simulink model "ASM_Traffic"  (R2026a)
settings: Solver=ode1  StartTime=SIM.tstart.v  StopTime=SIM.tend.v  FixedStep=SIM.StepSize.v
PostLoadFcn:
  | if any(exist('dsrtsu_mdlpostloadfcn', 'file') ~= 0), dsrtsu_mdlpostloadfcn('Execute', bdroot); end
  | try, asm_mdl_postloadfcn(bdroot, 'UpdateModel', 3600); catch, disp(lasterr); end,
InitFcn:
  | , if any(exist('rtifpga_mdlclblib', 'file') ~= 0), rtifpga_mdlclblib('Init', bdroot); end,
  | , if any(exist('dsmpb_private', 'file') ~= 0), dsmpb_private('dsmpb_mdlclblib', 'Init', bdroot); end,
model workspace (MAT data in the model file):
  asmReferencePath = [0 0.01 0.02 0.03 0.04 0.05 0.06 0.07 0.08 0.09 0.1 0.11 ... (350007 elements, 50001x7)]
  roadBounds : Simulink.Parameter (value not decoded)
  safetyAxes : Simulink.Parameter (value not decoded)
undefined symbols (not defined in the file): _to_, a0b2, ASM_BrakeHydraulics_DemoSystems, ASM_VehicleDynamics_DemoSystems, b98103fe8ad365046cd0, BrakeCircuit, controllerConfig, CPT, Crankshaft, DiscIntNeverNeededParam, dsmsi, FinalDriveAssembly, MDL, ModeSignals, mu, Pos_BrakePedal_Maneuver, rad, RefSignals, roadFamilyData, roadFamilyId, s_to_rpm, SIM, SoftECU, Suspension, Tire, Transmission
libraries: ASM_Traffic_lib x135, simulink x98, ASM_Utils_lib x77, ASM_VehicleDynamics_lib x70, ASM_Environment_lib x22, dsmpblib x20, dsmsilib x15, MDLD_Utils_lib x10, ASM_BrakeHydraulics_lib x3, sl_discontinuities x2
(part 41 of 65)

== system ASM_Traffic/Environment/Sensors/PlantModel/Object_Sensor_2D/SensorParameters ==
  2D_Sensors_Common_Signals : Subsystem
  Bus Creator : BusCreator  Inputs=8
  Demux{,1..6} (7 alike) : Demux  Outputs=3
  Mux{1..7} (7 alike) : Mux  Inputs=14
  OBJECT_SENSOR_2D_PARAMETERS_1 : ASM_Traffic_lib/Sensors/Object_Sensor_2D/OBJECT_SENSOR_2D_PARAMETERS  Tag=ASM_SUBCOMPONENT  Sw_Sensor_Enable=MDL.Traffic.Sensors.ObjectSensor2D_1.Sw_Sensor_Enable  Const_SensorIdx=MDL.Traffic.Sensors.ObjectSensor2D_1.Const_SensorIdx  Const_t_Offs_Sensor=MDL.Traffic.Sensors.ObjectSensor2D_1.Const_t_Offs_Sensor  Const_t_Cycle_Sensor=MDL.Traffic.Sensors.ObjectSensor2D_1.Const_t_Cycle_Sensor  Const_t_Delay_SensorOutput=MDL.Traffic.Sensors.ObjectSensor2D_1.Const_t_Delay_SensorOutput  Const_Pos_Sensor_Apex_CoorSys_V=MDL.Traffic.Sensors.ObjectSensor2D_1.Const_Pos_Sensor_Apex_CoorSys_V  Const_Angle_z_Orientation_Sensor_CoorSys_V=MDL.Traffic.Sensors.ObjectSensor2D_1.Const_Angle_z_Orientation_Sensor_CoorSys_V  Const_Angle_ScopeZone_Horizontal=MDL.Traffic.Sensors.ObjectSensor2D_1.Const_Angle_ScopeZone_Horizontal  Const_Length_ScopeZone=MDL.Traffic.Sensors.ObjectSensor2D_1.Const_Length_ScopeZone  Const_Num_SensorRays_Used=MDL.Traffic.Sensors.ObjectSensor2D_1.Const_Num_SensorRays_Used  Sw_Sensor_Detection_Mode=MDL.Traffic.Sensors.ObjectSensor2D_1.Sw_Sensor_Detection_Mode  Sw_Object_Detection_Mode=MDL.Traffic.Sensors.ObjectSensor2D_1.Sw_Object_Detection_Mode  ASMProperties=struct('Name','OBJECT_SENSOR_2D_PARAMETERS','Version','5.0','Library','ASM_Traffic_lib')  ASMInstanceName=object_sensor_2d_parameters  ASMInstanceID=1
  OBJECT_SENSOR_2D_PARAMETERS_2 : ASM_Traffic_lib/Sensors/Object_Sensor_2D/OBJECT_SENSOR_2D_PARAMETERS  Tag=ASM_SUBCOMPONENT  Sw_Sensor_Enable=MDL.Traffic.Sensors.ObjectSensor2D_2.Sw_Sensor_Enable  Const_SensorIdx=MDL.Traffic.Sensors.ObjectSensor2D_2.Const_SensorIdx  Const_t_Offs_Sensor=MDL.Traffic.Sensors.ObjectSensor2D_2.Const_t_Offs_Sensor  Const_t_Cycle_Sensor=MDL.Traffic.Sensors.ObjectSensor2D_2.Const_t_Cycle_Sensor  Const_t_Delay_SensorOutput=MDL.Traffic.Sensors.ObjectSensor2D_2.Const_t_Delay_SensorOutput  Const_Pos_Sensor_Apex_CoorSys_V=MDL.Traffic.Sensors.ObjectSensor2D_2.Const_Pos_Sensor_Apex_CoorSys_V  Const_Angle_z_Orientation_Sensor_CoorSys_V=MDL.Traffic.Sensors.ObjectSensor2D_2.Const_Angle_z_Orientation_Sensor_CoorSys_V  Const_Angle_ScopeZone_Horizontal=MDL.Traffic.Sensors.ObjectSensor2D_2.Const_Angle_ScopeZone_Horizontal  Const_Length_ScopeZone=MDL.Traffic.Sensors.ObjectSensor2D_2.Const_Length_ScopeZone  Const_Num_SensorRays_Used=MDL.Traffic.Sensors.ObjectSensor2D_2.Const_Num_SensorRays_Used  Sw_Sensor_Detection_Mode=MDL.Traffic.Sensors.ObjectSensor2D_2.Sw_Sensor_Detection_Mode  Sw_Object_Detection_Mode=MDL.Traffic.Sensors.ObjectSensor2D_2.Sw_Object_Detection_Mode  ASMProperties=struct('Name','OBJECT_SENSOR_2D_PARAMETERS','Version','5.0','Library','ASM_Traffic_lib')  ASMInstanceName=object_sensor_2d_parameters  ASMInstanceID=2
      settings: AttributesFormatString=Instance Name: %<ASMInstanceName>\nInstance ID: %<ASMInstanceID>
  OBJECT_SENSOR_2D_PARAMETERS_3 : ASM_Traffic_lib/Sensors/Object_Sensor_2D/OBJECT_SENSOR_2D_PARAMETERS  Tag=ASM_SUBCOMPONENT  Sw_Sensor_Enable=MDL.Traffic.Sensors.ObjectSensor2D_3.Sw_Sensor_Enable  Const_SensorIdx=MDL.Traffic.Sensors.ObjectSensor2D_3.Const_SensorIdx  Const_t_Offs_Sensor=MDL.Traffic.Sensors.ObjectSensor2D_3.Const_t_Offs_Sensor  Const_t_Cycle_Sensor=MDL.Traffic.Sensors.ObjectSensor2D_3.Const_t_Cycle_Sensor  Const_t_Delay_SensorOutput=MDL.Traffic.Sensors.ObjectSensor2D_3.Const_t_Delay_SensorOutput  Const_Pos_Sensor_Apex_CoorSys_V=MDL.Traffic.Sensors.ObjectSensor2D_3.Const_Pos_Sensor_Apex_CoorSys_V  Const_Angle_z_Orientation_Sensor_CoorSys_V=MDL.Traffic.Sensors.ObjectSensor2D_3.Const_Angle_z_Orientation_Sensor_CoorSys_V  Const_Angle_ScopeZone_Horizontal=MDL.Traffic.Sensors.ObjectSensor2D_3.Const_Angle_ScopeZone_Horizontal  Const_Length_ScopeZone=MDL.Traffic.Sensors.ObjectSensor2D_3.Const_Length_ScopeZone  Const_Num_SensorRays_Used=MDL.Traffic.Sensors.ObjectSensor2D_3.Const_Num_SensorRays_Used  Sw_Sensor_Detection_Mode=MDL.Traffic.Sensors.ObjectSensor2D_3.Sw_Sensor_Detection_Mode  Sw_Object_Detection_Mode=MDL.Traffic.Sensors.ObjectSensor2D_3.Sw_Object_Detection_Mode  ASMProperties=struct('Name','OBJECT_SENSOR_2D_PARAMETERS','Version','5.0','Library','ASM_Traffic_lib')  ASMInstanceName=object_sensor_2d_parameters  ASMInstanceID=3
      settings: AttributesFormatString=Instance Name: %<ASMInstanceName>\nInstance ID: %<ASMInstanceID>
  OBJECT_SENSOR_2D_PARAMETERS_4 : ASM_Traffic_lib/Sensors/Object_Sensor_2D/OBJECT_SENSOR_2D_PARAMETERS  Tag=ASM_SUBCOMPONENT  Sw_Sensor_Enable=MDL.Traffic.Sensors.ObjectSensor2D_4.Sw_Sensor_Enable  Const_SensorIdx=MDL.Traffic.Sensors.ObjectSensor2D_4.Const_SensorIdx  Const_t_Offs_Sensor=MDL.Traffic.Sensors.ObjectSensor2D_4.Const_t_Offs_Sensor  Const_t_Cycle_Sensor=MDL.Traffic.Sensors.ObjectSensor2D_4.Const_t_Cycle_Sensor  Const_t_Delay_SensorOutput=MDL.Traffic.Sensors.ObjectSensor2D_4.Const_t_Delay_SensorOutput  Const_Pos_Sensor_Apex_CoorSys_V=MDL.Traffic.Sensors.ObjectSensor2D_4.Const_Pos_Sensor_Apex_CoorSys_V  Const_Angle_z_Orientation_Sensor_CoorSys_V=MDL.Traffic.Sensors.ObjectSensor2D_4.Const_Angle_z_Orientation_Sensor_CoorSys_V  Const_Angle_ScopeZone_Horizontal=MDL.Traffic.Sensors.ObjectSensor2D_4.Const_Angle_ScopeZone_Horizontal  Const_Length_ScopeZone=MDL.Traffic.Sensors.ObjectSensor2D_4.Const_Length_ScopeZone  Const_Num_SensorRays_Used=MDL.Traffic.Sensors.ObjectSensor2D_4.Const_Num_SensorRays_Used  Sw_Sensor_Detection_Mode=MDL.Traffic.Sensors.ObjectSensor2D_4.Sw_Sensor_Detection_Mode  Sw_Object_Detection_Mode=MDL.Traffic.Sensors.ObjectSensor2D_4.Sw_Object_Detection_Mode  ASMProperties=struct('Name','OBJECT_SENSOR_2D_PARAMETERS','Version','5.0','Library','ASM_Traffic_lib')  ASMInstanceName=object_sensor_2d_parameters  ASMInstanceID=4
      settings: AttributesFormatString=Instance Name: %<ASMInstanceName>\nInstance ID: %<ASMInstanceID>
  OBJECT_SENSOR_2D_PARAMETERS_5 : ASM_Traffic_lib/Sensors/Object_Sensor_2D/OBJECT_SENSOR_2D_PARAMETERS  Tag=ASM_SUBCOMPONENT  Sw_Sensor_Enable=MDL.Traffic.Sensors.ObjectSensor2D_5.Sw_Sensor_Enable  Const_SensorIdx=MDL.Traffic.Sensors.ObjectSensor2D_5.Const_SensorIdx  Const_t_Offs_Sensor=MDL.Traffic.Sensors.ObjectSensor2D_5.Const_t_Offs_Sensor  Const_t_Cycle_Sensor=MDL.Traffic.Sensors.ObjectSensor2D_5.Const_t_Cycle_Sensor  Const_t_Delay_SensorOutput=MDL.Traffic.Sensors.ObjectSensor2D_5.Const_t_Delay_SensorOutput  Const_Pos_Sensor_Apex_CoorSys_V=MDL.Traffic.Sensors.ObjectSensor2D_5.Const_Pos_Sensor_Apex_CoorSys_V  Const_Angle_z_Orientation_Sensor_CoorSys_V=MDL.Traffic.Sensors.ObjectSensor2D_5.Const_Angle_z_Orientation_Sensor_CoorSys_V  Const_Angle_ScopeZone_Horizontal=MDL.Traffic.Sensors.ObjectSensor2D_5.Const_Angle_ScopeZone_Horizontal  Const_Length_ScopeZone=MDL.Traffic.Sensors.ObjectSensor2D_5.Const_Length_ScopeZone  Const_Num_SensorRays_Used=MDL.Traffic.Sensors.ObjectSensor2D_5.Const_Num_SensorRays_Used  Sw_Sensor_Detection_Mode=MDL.Traffic.Sensors.ObjectSensor2D_5.Sw_Sensor_Detection_Mode  Sw_Object_Detection_Mode=MDL.Traffic.Sensors.ObjectSensor2D_5.Sw_Object_Detection_Mode  ASMProperties=struct('Name','OBJECT_SENSOR_2D_PARAMETERS','Version','5.0','Library','ASM_Traffic_lib')  ASMInstanceName=object_sensor_2d_parameters  ASMInstanceID=5
      settings: AttributesFormatString=Instance Name: %<ASMInstanceName>\nInstance ID: %<ASMInstanceID>
  OBJECT_SENSOR_2D_PARAMETERS_6 : ASM_Traffic_lib/Sensors/Object_Sensor_2D/OBJECT_SENSOR_2D_PARAMETERS  Tag=ASM_SUBCOMPONENT  Sw_Sensor_Enable=MDL.Traffic.Sensors.ObjectSensor2D_6.Sw_Sensor_Enable  Const_SensorIdx=MDL.Traffic.Sensors.ObjectSensor2D_6.Const_SensorIdx  Const_t_Offs_Sensor=MDL.Traffic.Sensors.ObjectSensor2D_6.Const_t_Offs_Sensor  Const_t_Cycle_Sensor=MDL.Traffic.Sensors.ObjectSensor2D_6.Const_t_Cycle_Sensor  Const_t_Delay_SensorOutput=MDL.Traffic.Sensors.ObjectSensor2D_6.Const_t_Delay_SensorOutput  Const_Pos_Sensor_Apex_CoorSys_V=MDL.Traffic.Sensors.ObjectSensor2D_6.Const_Pos_Sensor_Apex_CoorSys_V  Const_Angle_z_Orientation_Sensor_CoorSys_V=MDL.Traffic.Sensors.ObjectSensor2D_6.Const_Angle_z_Orientation_Sensor_CoorSys_V  Const_Angle_ScopeZone_Horizontal=MDL.Traffic.Sensors.ObjectSensor2D_6.Const_Angle_ScopeZone_Horizontal  Const_Length_ScopeZone=MDL.Traffic.Sensors.ObjectSensor2D_6.Const_Length_ScopeZone  Const_Num_SensorRays_Used=MDL.Traffic.Sensors.ObjectSensor2D_6.Const_Num_SensorRays_Used  Sw_Sensor_Detection_Mode=MDL.Traffic.Sensors.ObjectSensor2D_6.Sw_Sensor_Detection_Mode  Sw_Object_Detection_Mode=MDL.Traffic.Sensors.ObjectSensor2D_6.Sw_Object_Detection_Mode  ASMProperties=struct('Name','OBJECT_SENSOR_2D_PARAMETERS','Version','5.0','Library','ASM_Traffic_lib')  ASMInstanceName=object_sensor_2d_parameters  ASMInstanceID=6
      settings: AttributesFormatString=Instance Name: %<ASMInstanceName>\nInstance ID: %<ASMInstanceID>
  OBJECT_SENSOR_2D_PARAMETERS_7 : ASM_Traffic_lib/Sensors/Object_Sensor_2D/OBJECT_SENSOR_2D_PARAMETERS  Tag=ASM_SUBCOMPONENT  Sw_Sensor_Enable=MDL.Traffic.Sensors.ObjectSensor2D_7.Sw_Sensor_Enable  Const_SensorIdx=MDL.Traffic.Sensors.ObjectSensor2D_7.Const_SensorIdx  Const_t_Offs_Sensor=MDL.Traffic.Sensors.ObjectSensor2D_7.Const_t_Offs_Sensor  Const_t_Cycle_Sensor=MDL.Traffic.Sensors.ObjectSensor2D_7.Const_t_Cycle_Sensor  Const_t_Delay_SensorOutput=MDL.Traffic.Sensors.ObjectSensor2D_7.Const_t_Delay_SensorOutput  Const_Pos_Sensor_Apex_CoorSys_V=MDL.Traffic.Sensors.ObjectSensor2D_7.Const_Pos_Sensor_Apex_CoorSys_V  Const_Angle_z_Orientation_Sensor_CoorSys_V=MDL.Traffic.Sensors.ObjectSensor2D_7.Const_Angle_z_Orientation_Sensor_CoorSys_V  Const_Angle_ScopeZone_Horizontal=MDL.Traffic.Sensors.ObjectSensor2D_7.Const_Angle_ScopeZone_Horizontal  Const_Length_ScopeZone=MDL.Traffic.Sensors.ObjectSensor2D_7.Const_Length_ScopeZone  Const_Num_SensorRays_Used=MDL.Traffic.Sensors.ObjectSensor2D_7.Const_Num_SensorRays_Used  Sw_Sensor_Detection_Mode=MDL.Traffic.Sensors.ObjectSensor2D_7.Sw_Sensor_Detection_Mode  Sw_Object_Detection_Mode=MDL.Traffic.Sensors.ObjectSensor2D_7.Sw_Object_Detection_Mode  ASMProperties=struct('Name','OBJECT_SENSOR_2D_PARAMETERS','Version','5.0','Library','ASM_Traffic_lib')  ASMInstanceName=object_sensor_2d_parameters  ASMInstanceID=7
      settings: AttributesFormatString=Instance Name: %<ASMInstanceName>\nInstance ID: %<ASMInstanceID>
  Vector Concatenate : Concatenate  NumInputs=7  Mode=Multidimensional array  ConcatenateDimension=2
  Sensor_Data[] : Outport  VectorParamsAs1DForOutWhenUnconnected=off
  tag scope: ASMBUS_Environment_Traffic_2DObjSensor_Parameter=scoped
  wires:
  [ASMBUS_Environment_Traffic_2DObjSensor2_Parameter] -> Bus Creator/3  "Sensor2"
  [ASMBUS_Environment_Traffic_2DObjSensor3_Parameter] -> Bus Creator/4  "Sensor3"
  [ASMBUS_Environment_Traffic_2DObjSensor1_Parameter] -> Bus Creator/2  "Sensor1"
  Bus Creator/1 -> [ASMBUS_Environment_Traffic_2DObjSensor_Parameter]
  [ASMBUS_Environment_Traffic_2DObjSensor4_Parameter] -> Bus Creator/5  "Sensor4"
  [ASMBUS_Environment_Traffic_2DObjSensor6_Parameter] -> Bus Creator/7  "Sensor6"
  [ASMBUS_Environment_Traffic_2DObjSensor5_Parameter] -> Bus Creator/6  "Sensor5"
  [ASMBUS_Environment_Traffic_2DObjSensor7_Parameter] -> Bus Creator/8  "Sensor7"
  OBJECT_SENSOR_2D_PARAMETERS_3/13 -> Mux3/14
  OBJECT_SENSOR_2D_PARAMETERS_4/13 -> Mux4/14
  OBJECT_SENSOR_2D_PARAMETERS_7/13 -> Mux7/14
  OBJECT_SENSOR_2D_PARAMETERS_6/13 -> Mux6/14
  OBJECT_SENSOR_2D_PARAMETERS_5/13 -> Mux5/14
  OBJECT_SENSOR_2D_PARAMETERS_2/13 -> Mux2/14
  OBJECT_SENSOR_2D_PARAMETERS_1/13 -> Mux1/14
  OBJECT_SENSOR_2D_PARAMETERS_7/12 -> Mux7/13
  OBJECT_SENSOR_2D_PARAMETERS_7/11 -> Mux7/12
  OBJECT_SENSOR_2D_PARAMETERS_7/10 -> Mux7/11
  OBJECT_SENSOR_2D_PARAMETERS_7/9 -> Mux7/10
  OBJECT_SENSOR_2D_PARAMETERS_7/8 -> Mux7/9
  OBJECT_SENSOR_2D_PARAMETERS_7/6 -> Mux7/5
  OBJECT_SENSOR_2D_PARAMETERS_7/5 -> Mux7/4
  OBJECT_SENSOR_2D_PARAMETERS_7/4 -> Mux7/3
  OBJECT_SENSOR_2D_PARAMETERS_7/3 -> Mux7/2
  OBJECT_SENSOR_2D_PARAMETERS_7/2 -> Mux7/1
  Demux6/3 -> Mux7/8
  Demux6/2 -> Mux7/7
  Demux6/1 -> Mux7/6
  Mux7/1 -> Vector Concatenate/7
  OBJECT_SENSOR_2D_PARAMETERS_7/7 -> Demux6/1
  OBJECT_SENSOR_2D_PARAMETERS_6/12 -> Mux6/13
  OBJECT_SENSOR_2D_PARAMETERS_6/11 -> Mux6/12
  OBJECT_SENSOR_2D_PARAMETERS_6/10 -> Mux6/11
  OBJECT_SENSOR_2D_PARAMETERS_6/9 -> Mux6/10
  OBJECT_SENSOR_2D_PARAMETERS_6/8 -> Mux6/9
  OBJECT_SENSOR_2D_PARAMETERS_6/6 -> Mux6/5
  OBJECT_SENSOR_2D_PARAMETERS_6/5 -> Mux6/4
  OBJECT_SENSOR_2D_PARAMETERS_6/4 -> Mux6/3
  OBJECT_SENSOR_2D_PARAMETERS_6/3 -> Mux6/2
  OBJECT_SENSOR_2D_PARAMETERS_6/2 -> Mux6/1
  Demux5/3 -> Mux6/8
  Demux5/2 -> Mux6/7
  Demux5/1 -> Mux6/6
  Mux6/1 -> Vector Concatenate/6
  OBJECT_SENSOR_2D_PARAMETERS_6/7 -> Demux5/1
  OBJECT_SENSOR_2D_PARAMETERS_5/12 -> Mux5/13
  OBJECT_SENSOR_2D_PARAMETERS_5/11 -> Mux5/12
  OBJECT_SENSOR_2D_PARAMETERS_5/10 -> Mux5/11
  OBJECT_SENSOR_2D_PARAMETERS_5/9 -> Mux5/10
  OBJECT_SENSOR_2D_PARAMETERS_5/8 -> Mux5/9
  OBJECT_SENSOR_2D_PARAMETERS_5/6 -> Mux5/5
  OBJECT_SENSOR_2D_PARAMETERS_5/5 -> Mux5/4
  OBJECT_SENSOR_2D_PARAMETERS_5/4 -> Mux5/3
  OBJECT_SENSOR_2D_PARAMETERS_5/3 -> Mux5/2
  OBJECT_SENSOR_2D_PARAMETERS_5/2 -> Mux5/1
  Demux4/3 -> Mux5/8
  Demux4/2 -> Mux5/7
  Demux4/1 -> Mux5/6
  Mux5/1 -> Vector Concatenate/5
  OBJECT_SENSOR_2D_PARAMETERS_5/7 -> Demux4/1
  OBJECT_SENSOR_2D_PARAMETERS_4/12 -> Mux4/13
  OBJECT_SENSOR_2D_PARAMETERS_4/11 -> Mux4/12
  OBJECT_SENSOR_2D_PARAMETERS_4/10 -> Mux4/11
  OBJECT_SENSOR_2D_PARAMETERS_4/9 -> Mux4/10
  OBJECT_SENSOR_2D_PARAMETERS_4/8 -> Mux4/9
  OBJECT_SENSOR_2D_PARAMETERS_4/6 -> Mux4/5
  OBJECT_SENSOR_2D_PARAMETERS_4/5 -> Mux4/4
  OBJECT_SENSOR_2D_PARAMETERS_4/4 -> Mux4/3
  OBJECT_SENSOR_2D_PARAMETERS_4/3 -> Mux4/2
  OBJECT_SENSOR_2D_PARAMETERS_4/2 -> Mux4/1
  Demux3/3 -> Mux4/8
  Demux3/2 -> Mux4/7
  Demux3/1 -> Mux4/6
  Mux4/1 -> Vector Concatenate/4
  OBJECT_SENSOR_2D_PARAMETERS_4/7 -> Demux3/1
  OBJECT_SENSOR_2D_PARAMETERS_7/1 -> [ASMBUS_Environment_Traffic_2DObjSensor7_Parameter]
  OBJECT_SENSOR_2D_PARAMETERS_6/1 -> [ASMBUS_Environment_Traffic_2DObjSensor6_Parameter]
  OBJECT_SENSOR_2D_PARAMETERS_5/1 -> [ASMBUS_Environment_Traffic_2DObjSensor5_Parameter]
  OBJECT_SENSOR_2D_PARAMETERS_4/1 -> [ASMBUS_Environment_Traffic_2DObjSensor4_Parameter]
  OBJECT_SENSOR_2D_PARAMETERS_3/12 -> Mux3/13
  OBJECT_SENSOR_2D_PARAMETERS_2/12 -> Mux2/13
  OBJECT_SENSOR_2D_PARAMETERS_1/12 -> Mux1/13
  OBJECT_SENSOR_2D_PARAMETERS_3/11 -> Mux3/12
  OBJECT_SENSOR_2D_PARAMETERS_3/10 -> Mux3/11
  OBJECT_SENSOR_2D_PARAMETERS_3/9 -> Mux3/10
  OBJECT_SENSOR_2D_PARAMETERS_3/8 -> Mux3/9
  OBJECT_SENSOR_2D_PARAMETERS_3/6 -> Mux3/5
  OBJECT_SENSOR_2D_PARAMETERS_3/5 -> Mux3/4
  OBJECT_SENSOR_2D_PARAMETERS_3/4 -> Mux3/3
  OBJECT_SENSOR_2D_PARAMETERS_3/3 -> Mux3/2
  OBJECT_SENSOR_2D_PARAMETERS_3/2 -> Mux3/1
  Demux2/3 -> Mux3/8
  Demux2/2 -> Mux3/7
  Demux2/1 -> Mux3/6
  Mux3/1 -> Vector Concatenate/3
  OBJECT_SENSOR_2D_PARAMETERS_3/7 -> Demux2/1
  OBJECT_SENSOR_2D_PARAMETERS_3/1 -> [ASMBUS_Environment_Traffic_2DObjSensor3_Parameter]
  OBJECT_SENSOR_2D_PARAMETERS_2/11 -> Mux2/12
  OBJECT_SENSOR_2D_PARAMETERS_2/10 -> Mux2/11
  OBJECT_SENSOR_2D_PARAMETERS_2/9 -> Mux2/10
  OBJECT_SENSOR_2D_PARAMETERS_2/8 -> Mux2/9
  OBJECT_SENSOR_2D_PARAMETERS_2/6 -> Mux2/5
  OBJECT_SENSOR_2D_PARAMETERS_2/5 -> Mux2/4
  OBJECT_SENSOR_2D_PARAMETERS_2/4 -> Mux2/3
  OBJECT_SENSOR_2D_PARAMETERS_2/3 -> Mux2/2
  OBJECT_SENSOR_2D_PARAMETERS_2/2 -> Mux2/1
  Demux1/3 -> Mux2/8
  Demux1/2 -> Mux2/7
  Demux1/1 -> Mux2/6
  Mux2/1 -> Vector Concatenate/2
  OBJECT_SENSOR_2D_PARAMETERS_2/7 -> Demux1/1
  OBJECT_SENSOR_2D_PARAMETERS_2/1 -> [ASMBUS_Environment_Traffic_2DObjSensor2_Parameter]
  OBJECT_SENSOR_2D_PARAMETERS_1/11 -> Mux1/12
  OBJECT_SENSOR_2D_PARAMETERS_1/10 -> Mux1/11
  OBJECT_SENSOR_2D_PARAMETERS_1/9 -> Mux1/10
  OBJECT_SENSOR_2D_PARAMETERS_1/8 -> Mux1/9
  OBJECT_SENSOR_2D_PARAMETERS_1/6 -> Mux1/5
  OBJECT_SENSOR_2D_PARAMETERS_1/5 -> Mux1/4
  OBJECT_SENSOR_2D_PARAMETERS_1/4 -> Mux1/3
  OBJECT_SENSOR_2D_PARAMETERS_1/3 -> Mux1/2
  OBJECT_SENSOR_2D_PARAMETERS_1/2 -> Mux1/1
  Demux/3 -> Mux1/8
  Demux/2 -> Mux1/7
  Demux/1 -> Mux1/6
  Vector Concatenate/1 -> Sensor_Data[]/1, 2D_Sensors_Common_Signals/1(Sensor_Data[])
  Mux1/1 -> Vector Concatenate/1
  OBJECT_SENSOR_2D_PARAMETERS_1/7 -> Demux/1
  OBJECT_SENSOR_2D_PARAMETERS_1/1 -> [ASMBUS_Environment_Traffic_2DObjSensor1_Parameter]
  2D_Sensors_Common_Signals/1(2D_Sensors_Common_Signals) -> Bus Creator/1

== system ASM_Traffic/Environment/Sensors/PlantModel/Object_Sensor_3D/ASMSignalCollector ==
  Bus Creator : BusCreator  Inputs=6
  Bus Creator1 : BusCreator  Inputs=8
  Bus Creator2 : BusCreator  Inputs=8
  Bus Creator3 : BusCreator  Inputs=8
  Bus Selector : BusSelector  OutputSignals=SensorIndex,Info,SensorOutput,SensorTimeStamp
  Bus Selector1 : BusSelector  OutputSignals=SensorIndex,Info,SensorOutput,SensorTimeStamp
  Bus Selector{7..10} (4 alike) : BusSelector  OutputSignals=Sensor2
  Bus Selector{11..14} (4 alike) : BusSelector  OutputSignals=Sensor3
  Bus Selector2 : BusSelector  OutputSignals=SensorIndex,Info,SensorOutput,SensorTimeStamp
  Bus Selector{3..6} (4 alike) : BusSelector  OutputSignals=Sensor1
  Rename : Subsystem
  Rename1 : Subsystem
  Rename2 : Subsystem
  Rename3 : Subsystem
  Rename4 : Subsystem
  Rename5 : Subsystem
  Rename6 : Subsystem
  Rename7 : Subsystem
  Rename8 : Subsystem
  Sensor_1_Info : Subsystem
  Sensor_2_Info : Subsystem
  Sensor_3_Info : Subsystem
  tag scope: ASMBUS_Environment_Trafffic_Sensors_Object_Sensor_3D=scoped
  wires:
  Bus Selector11/1 -> Bus Selector2/1  "<Sensor3>"
  Rename8/1(Out1) -> Bus Creator3/8  "ObjectData"
  Bus Selector14/1 -> Rename8/1(In1)  "<Sensor3>"
  Rename7/1(Out1) -> Bus Creator3/7  "CustomPoints"
  Bus Selector13/1 -> Rename7/1(In1)  "<Sensor3>"
  Bus Selector12/1 -> Rename6/1(In1)  "<Sensor3>"
  Rename6/1(Out1) -> Bus Creator3/6  "RadarEffects"
  Rename3/1(Out1) -> Bus Creator2/6  "RadarEffects"
  Rename4/1(Out1) -> Bus Creator2/7  "CustomPoints"
  Rename5/1(Out1) -> Bus Creator2/8  "ObjectData"
  Bus Selector10/1 -> Rename5/1(In1)  "<Sensor2>"
  Bus Selector9/1 -> Rename4/1(In1)  "<Sensor2>"
  Bus Selector7/1 -> Bus Selector1/1  "<Sensor2>"
  Bus Selector8/1 -> Rename3/1(In1)  "<Sensor2>"
  Rename2/1(Out1) -> Bus Creator1/8  "ObjectData"
  Bus Selector6/1 -> Rename2/1(In1)  "<Sensor1>"
  Rename1/1(Out1) -> Bus Creator1/7  "CustomPoints"
  Bus Selector5/1 -> Rename1/1(In1)  "<Sensor1>"
  Rename/1(Out1) -> Bus Creator1/6  "RadarEffects"
  Bus Selector4/1 -> Rename/1(In1)  "<Sensor1>"
  [ASMBUS_Environment_Traffic_3DObjSensor_ObjectData] -> Bus Selector14/1
  [ASMBUS_Environment_Traffic_3DObjSensor_CustomPoints] -> Bus Selector13/1
  [ASMBUS_Environment_Traffic_3DObjSensor_RadarEffects] -> Bus Selector12/1
  [ASMBUS_Environment_Traffic_3DObjSensor_SensorSignals] -> Bus Selector11/1
  [ASMBUS_Environment_Traffic_3DObjSensor_RadarEffects] -> Bus Selector4/1
  [ASMBUS_Environment_Traffic_3DObjSensor_SensorSignals] -> Bus Selector3/1
  [ASMBUS_Environment_Traffic_3DObjSensor_ObjectData] -> Bus Selector10/1
  [ASMBUS_Environment_Traffic_3DObjSensor_ObjectData] -> Bus Selector6/1
  [ASMBUS_Environment_Traffic_3DObjSensors_Boundingboxes] -> Bus Creator/6
  Sensor_3_Info/1(Info) -> Bus Creator3/3  "Info"
  Sensor_2_Info/1(Info) -> Bus Creator2/3  "Info"
  [ASMBUS_Environment_Traffic_3DObjSensor_SensorSignals_Status] -> Sensor_3_Info/2(Sensor_Status), Sensor_2_Info/2(Sensor_Status), Sensor_1_Info/2(Sfcn_Status)
  Sensor_1_Info/1(Info) -> Bus Creator1/3  "Info"
  Bus Selector/2 -> Sensor_1_Info/1(Sensor_Info)  "<Info>"
  [ASMBUS_Environment_Traffic_3DObjSensor_RadarEffects] -> Bus Selector8/1
  [ASMBUS_Environment_Traffic_3DObjSensor_CustomPoints] -> Bus Selector9/1
  [ASMBUS_Environment_Traffic_3DObjSensor_CustomPoints] -> Bus Selector5/1
  [ASMBUS_Environment_Traffic_SamplePulse] -> Bus Creator/1  "Sample_Pulse"
  [ASMBUS_Environment_Traffic_SensorScheduler] -> Bus Creator/2  "Sensor_Scheduler"
  Bus Selector/3 -> Bus Creator1/4  "<SensorOutput>"
  Bus Selector2/3 -> Bus Creator3/4  "<SensorOutput>"
  Bus Selector2/2 -> Sensor_3_Info/1(Sensor_Info)  "<Info>"
  Bus Selector1/3 -> Bus Creator2/4  "<SensorOutput>"
  Bus Selector1/2 -> Sensor_2_Info/1(Sensor_Info)  "<Info>"
  Bus Selector1/1 -> Bus Creator2/2  "<SensorIndex>"
  Bus Selector/1 -> Bus Creator1/2  "<SensorIndex>"
  [ASMBUS_Environment_Traffic_3DObjSensor3_Parameters] -> Bus Creator3/1  "Parameter"
  [ASMBUS_Environment_Traffic_3DObjSensor2_Parameters] -> Bus Creator2/1  "Parameter"
  [ASMBUS_Environment_Traffic_3DObjSensor1_Parameters] -> Bus Creator1/1  "Parameter"
  Bus Selector2/1 -> Bus Creator3/2  "<SensorIndex>"
  Bus Creator3/1 -> Bus Creator/5  "Sensor_3_Rear"
  Bus Creator2/1 -> Bus Creator/4  "Sensor_2_Front_Mid"
  Bus Creator1/1 -> Bus Creator/3  "Sensor_1_Front_Long"
  [ASMBUS_Environment_Traffic_3DObjSensor_SensorSignals] -> Bus Selector7/1
  Bus Selector3/1 -> Bus Selector/1  "<Sensor1>"
  Bus Creator/1 -> [ASMBUS_Environment_Trafffic_Sensors_Object_Sensor_3D]  "Object_Sensor_3D"
  Bus Selector/4 -> Bus Creator1/5  "<SensorTimeStamp>"
  Bus Selector1/4 -> Bus Creator2/5  "<SensorTimeStamp>"
  Bus Selector2/4 -> Bus Creator3/5  "<SensorTimeStamp>"

== system ASM_Traffic/Environment/Sensors/PlantModel/Object_Sensor_3D/CustomPoints ==
  Enable[0Off|1On] : Inport
  SensorMapping_Data[] : Inport  Port=2
  SensorData[] : Inport  Port=3
  Bus Creator : BusCreator  Inputs=3
  Demux : Demux  Outputs=[4,4,4]
  Sensor1 : Subsystem
  Sensor2 : Subsystem
  Sensor3 : Subsystem
  tag scope: ASMBUS_Environment_Traffic_3DObjSensor_CustomPoints=scoped
  wires:
  Bus Creator/1 -> [ASMBUS_Environment_Traffic_3DObjSensor_CustomPoints]
  Sensor3/1(CustomPoints_Signals[]) -> Bus Creator/3  "Sensor3"
  Sensor2/1(CustomPoints_Signals[]) -> Bus Creator/2  "Sensor2"
  Sensor1/1(CustomPoints_Signals[]) -> Bus Creator/1  "Sensor1"
  Enable[0Off|1On]/1 -> Sensor1/1(Enable[0|1]), Sensor2/1(Enable[0|1]), Sensor3/1(Enable[0|1])
  SensorData[]/1 -> Sensor1/3(SensorData[]), Sensor2/3(SensorData[]), Sensor3/3(SensorData[])
  Demux/3 -> Sensor3/2(SensorMapping_Data[])
  Demux/2 -> Sensor2/2(SensorMapping_Data[])
  Demux/1 -> Sensor1/2(SensorMapping_Data[])
  SensorMapping_Data[]/1 -> Demux/1

== system ASM_Traffic/Environment/Sensors/PlantModel/Object_Sensor_3D/Enable_Object_Sensor_3D ==
  Enable_In[0Off|1On] : Inport
  Constant : Constant  Value=0.5  SampleTime=-1
  Constant1 : Constant  SampleTime=-1
  Constant2 : Constant  Value=0  SampleTime=-1
  Enable_Sensor : Gain
  Multiport Switch : MultiPortSwitch  DataPortOrder=Zero-based contiguous  Inputs=2  zeroidx=on  SaturateOnIntegerOverflow=off  InputSameDT=off
  Relational Operator : RelationalOperator  Operator=>  OutDataTypeStr=boolean  InputSameDT=off
  Enable_Out[0Off|1On] : Outport  VectorParamsAs1DForOutWhenUnconnected=off
  wires:
  Constant2/1 -> Multiport Switch/2
  Constant1/1 -> Multiport Switch/3
  Constant/1 -> Relational Operator/2
  Multiport Switch/1 -> Enable_Out[0Off|1On]/1
  Relational Operator/1 -> Multiport Switch/1
  Enable_Sensor/1 -> Relational Operator/1
  Enable_In[0Off|1On]/1 -> Enable_Sensor/1

== system ASM_Traffic/Environment/Sensors/PlantModel/Object_Sensor_3D/ObjectData ==
  Traffic_Signals : Inport
  Road_Signals : Inport  Port=2
  BoundingBoxData_CoorSys_E : Subsystem
  Bus Creator : BusCreator  Inputs=3
  Bus Selector1 : BusSelector  OutputSignals=SensorOutput.Object_ID[],SensorOutput.Object_Type[]
  Bus Selector2 : BusSelector  OutputSignals=SensorOutput.Object_ID[],SensorOutput.Object_Type[]
  Bus Selector3 : BusSelector  OutputSignals=SensorOutput.Object_ID[],SensorOutput.Object_Type[]
  Bus Selector4 : BusSelector  OutputSignals=Sensor_1_Front_Long,Sensor_2_Front_Mid,Sensor_3_Rear
  Sensor1 : Subsystem
  Sensor2 : Subsystem
  Sensor3 : Subsystem
  Terminator{1..9} (9 alike) : Terminator
  avoid_incomplete_trace2source : Subsystem
  avoid_incomplete_trace2source1 : Subsystem
  avoid_incomplete_trace2source2 : Subsystem
  avoid_incomplete_trace2source3 : Subsystem
  avoid_incomplete_trace2source4 : Subsystem
  avoid_incomplete_trace2source5 : Subsystem
  tag scope: ASMBUS_Environment_Traffic_3DObjSensor_ObjectData=scoped
  wires:
  avoid_incomplete_trace2source5/1(Out1) -> Sensor3/2(Object_Type[])
  avoid_incomplete_trace2source4/1(Out1) -> Sensor3/1(Object_ID[])
  avoid_incomplete_trace2source2/1(Out1) -> Sensor2/1(Object_ID[])
  avoid_incomplete_trace2source3/1(Out1) -> Sensor2/2(Object_Type[])
  avoid_incomplete_trace2source1/1(Out1) -> Sensor1/2(Object_Type[])
  avoid_incomplete_trace2source/1(Out1) -> Sensor1/1(Object_ID[])
  Bus Creator/1 -> [ASMBUS_Environment_Traffic_3DObjSensor_ObjectData]
  Sensor3/1(ASMSignalBus) -> Bus Creator/3  "Sensor3"
  Sensor2/1(ASMSignalBus) -> Bus Creator/2  "Sensor2"
  Sensor1/1(ASMSignalBus) -> Bus Creator/1  "Sensor1"
  [ASMBUS_Environment_Trafffic_Sensors_Object_Sensor_3D] -> Bus Selector4/1
  Sensor3/3(Object_Properties_Box[]) -> Terminator8/1
  Sensor3/2(Object_Position[]) -> Terminator7/1
  Sensor3/4(Object_Custom_Values[]) -> Terminator9/1
  Bus Selector3/1 -> avoid_incomplete_trace2source4/1(In1)  "<Object_ID[]>"
  Bus Selector3/2 -> avoid_incomplete_trace2source5/1(In1)  "<Object_Type[]>"
  Bus Selector4/3 -> BoundingBoxData_CoorSys_E/5(Sensor3_Signals[]), Bus Selector3/1  "<Sensor_3_Rear>"
  Bus Selector4/2 -> BoundingBoxData_CoorSys_E/4(Sensor2_Signals[]), Bus Selector2/1  "<Sensor_2_Front_Mid>"
  Bus Selector2/2 -> avoid_incomplete_trace2source3/1(In1)  "<Object_Type[]>"
  Bus Selector2/1 -> avoid_incomplete_trace2source2/1(In1)  "<Object_ID[]>"
  Sensor2/4(Object_Custom_Values[]) -> Terminator6/1
  Sensor2/2(Object_Position[]) -> Terminator1/1
  Sensor2/3(Object_Properties_Box[]) -> Terminator2/1
  Bus Selector4/1 -> BoundingBoxData_CoorSys_E/3(Sensor1_Signals[]), Bus Selector1/1  "<Sensor_1_Front_Long>"
  Road_Signals/1 -> Sensor2/4(Road_Signals), Sensor3/4(Road_Signals), BoundingBoxData_CoorSys_E/2(Road_Signals), Sensor1/4(Road_Signals)
  Traffic_Signals/1 -> Sensor2/3(Traffic_Signals), BoundingBoxData_CoorSys_E/1(Traffic_Signals), Sensor3/3(Traffic_Signals), Sensor1/3(Traffic_Signals)
  Bus Selector1/2 -> avoid_incomplete_trace2source1/1(In1)  "<Object_Type[]>"
  Sensor1/3(Object_Properties_Box[]) -> Terminator4/1
  Sensor1/2(Object_Position[]) -> Terminator3/1
  Bus Selector1/1 -> avoid_incomplete_trace2source/1(In1)  "<Object_ID[]>"
  Sensor1/4(Object_Custom_Values[]) -> Terminator5/1

== system ASM_Traffic/Environment/Sensors/PlantModel/Object_Sensor_3D/RadarEffects ==
  Enable_Init[0Off|1On] : Inport
  Enable[0Off|1On] : Inport  Port=2
  SensorMapping_Data[] : Inport  Port=3
  SensorData[] : Inport  Port=4
  Angle_Vehicle_CoorSys_E[x;y;z][deg] : Inport  Port=5
  Pos_Vehicle_CoorSys_E[x;y;z][m] : Inport  Port=6
  Bus Creator : BusCreator  Inputs=3
  Data Type Conversion : DataTypeConversion  OutDataTypeStr=double  SaturateOnIntegerOverflow=off  RndMeth=Floor
  Demux1 : Demux  Outputs=[4,4,4]
  Hit Crossing : HitCross  HitCrossingOffset=0.5  HitCrossingDirection=rising
  Sensor1 : Subsystem
  Sensor2 : Subsystem
  Sensor3 : Subsystem
  tag scope: ASMBUS_Environment_Traffic_3DObjSensor_RadarEffects=scoped
  wires:
  Bus Creator/1 -> [ASMBUS_Environment_Traffic_3DObjSensor_RadarEffects]
  Hit Crossing/1 -> Data Type Conversion/1
  Data Type Conversion/1 -> Sensor1/1(Reset[]), Sensor2/1(Reset[]), Sensor3/1(Reset[])
  Enable_Init[0Off|1On]/1 -> Hit Crossing/1
  Sensor3/1(RadarEffect_Signals[]) -> Bus Creator/3  "Sensor3"
  Demux1/3 -> Sensor3/3(SensorMapping_Data[])
  Demux1/2 -> Sensor2/3(SensorMapping_Data[])
  Sensor2/1(RadarEffect_Signals[]) -> Bus Creator/2  "Sensor2"
  Sensor1/1(RadarEffect_Signals[]) -> Bus Creator/1  "Sensor1"
  Pos_Vehicle_CoorSys_E[x;y;z][m]/1 -> Sensor1/6(Pos_Vehicle_CoorSys_E[x;y;z][m]), Sensor2/6(Pos_Vehicle_CoorSys_E[x;y;z][m]), Sensor3/6(Pos_Vehicle_CoorSys_E[x;y;z][m])
  Angle_Vehicle_CoorSys_E[x;y;z][deg]/1 -> Sensor1/5(Angle_Vehicle_CoorSys_E[x;y;z][deg]), Sensor2/5(Angle_Vehicle_CoorSys_E[x;y;z][deg]), Sensor3/5(Angle_Vehicle_CoorSys_E[x;y;z][deg])
  Demux1/1 -> Sensor1/3(SensorMapping_Data[])
  SensorMapping_Data[]/1 -> Demux1/1
  SensorData[]/1 -> Sensor3/4(Sensor_Data[]), Sensor2/4(Sensor_Data[]), Sensor1/4(Sensor_Data[])
  Enable[0Off|1On]/1 -> Sensor1/2(Enable[0|1]), Sensor2/2(Enable[0|1]), Sensor3/2(Enable[0|1])

== system ASM_Traffic/Environment/Sensors/PlantModel/Object_Sensor_3D/ScheduleAndCalculateSensor ==
  Enable_Init[0Off|1On] : Inport
  Sensor_Data[] : Inport  Port=2
  Enable[0Off|1On] : Inport  Port=3
  Traffic_Signals : Inport  Port=4
  Interface_In : Inport  Port=5
  Road_Signals : Inport  Port=6
  Sensor_Time_Base[s] : Inport  Port=7
  Bus Selector : BusSelector  OutputSignals=ExternalModel.Angle_Vehicle_CoorSys_E[x;y;z][deg],ExternalModel.Pos_Vehicle_CoorSys_E[x;y;z][m]
  Bus Selector1 : BusSelector  OutputSignals=Info.Flag_Sensor_Init_Ready[0|1]  OutputAsBus=on
  Bus Selector2 : BusSelector  OutputSignals=Plant.ObjectParameters.TrafficObjects.TrafficObjectsState[]
  Bus Selector4 : BusSelector  OutputSignals=Plant.TrafficObject_Data[]  OutputAsBus=on
  Bus Selector5 : BusSelector  OutputSignals=Plant.Traffic_Signals_toEnvironment.Flag_FellowUsed[0|1],Plant.Traffic_Signals_toEnvironment.v_Fellows[x;y;z][km|h]
  Bus Selector6 : BusSelector  OutputSignals=Plant.Traffic_Signals_toEnvironment
  Bus to Vector : BusToVector
  GetFellowPositionVector : Subsystem
  GetObjectSignals : Subsystem
  Mux : Mux  Inputs=2
  OBJECT_SENSOR_3D_CALCULATION : ASM_Traffic_lib/Sensors/Object_Sensor_3D/OBJECT_SENSOR_3D_CALCULATION  Tag=ASM_SUBCOMPONENT  Const_Sensor_Output_Dimension=MDL.Traffic.Sensors.ObjectSensor3D_Calculation.Const_Sensor_Output_Dimension  Sw_Enable_Static_Objects=MDL.Traffic.Sensors.ObjectSensor3D_Calculation.Sw_Enable_Static_Objects  Sw_Output_Mode=MDL.Traffic.Sensors.ObjectSensor3D_Calculation.Sw_Output_Mode  StepSize=SIM.StepSize  ASMProperties=struct('Name','OBJECT_SENSOR_3D_CALCULATION','Version','13.0','Library','ASM_Traffic_lib')  ASMInstanceName=object_sensor_3d_calculation  ASMInstanceID=1
  OBJECT_SENSOR_3D_PARAM_SELECTION : ASM_Traffic_lib/Sensors/Object_Sensor_3D/OBJECT_SENSOR_3D_PARAM_SELECTION  ASMProperties=struct('Name','OBJECT_SENSOR_3D_PARAM_SELECTION','Version','4.0','Library','ASM_Traffic_lib')  ASMInstanceName=object_sensor_3d_param_selection  ASMInstanceID=1
  OBJECT_SENSOR_3D_PARAM_VECTORIZATION : ASM_Traffic_lib/Sensors/Object_Sensor_3D/OBJECT_SENSOR_3D_PARAM_VECTORIZATION  ASMProperties=struct('Name','OBJECT_SENSOR_3D_PARAM_VECTORIZATION','Version','4.0','Library','ASM_Traffic_lib')  ASMInstanceName=object_sensor_3d_param_vectorization  ASMInstanceID=1
  SAMPLE_PULSE : ASM_Traffic_lib/Sensors/Scheduling/SAMPLE_PULSE  Tag=ASM_SUBCOMPONENT  Sw_SamplePulse=MDL.Traffic.Sensors.SamplePulse.Sw_SamplePulse  Const_t_Offs_Pulse=MDL.Traffic.Sensors.SamplePulse.Const_t_Offs_Pulse  Const_t_Cycle_Pulse=MDL.Traffic.Sensors.SamplePulse.Const_t_Cycle_Pulse  StepSize=SIM.StepSize  ASMProperties=struct('Name','SAMPLE_PULSE','Version','3.0','Library','ASM_Traffic_lib')  ASMInstanceName=sample_pulse  ASMInstanceID=1
  SENSOR_SCHEDULER : ASM_Traffic_lib/Sensors/Scheduling/SENSOR_SCHEDULER  StepSize=SIM.StepSize  ASMProperties=struct('Name','SENSOR_SCHEDULER','Version','4.0','Library','ASM_Traffic_lib')  ASMInstanceName=sensor_scheduler  ASMInstanceID=1
  SampleAndHold : Subsystem  TreatAsAtomicUnit=on
  Terminator{1..4,7} (5 alike) : Terminator
  SensorMapping_Data[] : Outport  VectorParamsAs1DForOutWhenUnconnected=off
  SensorSignals : Outport  Port=2  VectorParamsAs1DForOutWhenUnconnected=off
  SensorData[] : Outport  Port=3  VectorParamsAs1DForOutWhenUnconnected=off
  Angle_Vehicle_CoorSys_E_Sampled[x,y;z][deg] : Outport  Port=4  VectorParamsAs1DForOutWhenUnconnected=off
  Pos_Vehicle_CoorSys_E_Sampled[x,y;z][m] : Outport  Port=5  VectorParamsAs1DForOutWhenUnconnected=off
  Init_Ready[0Off|1On] : Outport  Port=6  VectorParamsAs1DForOutWhenUnconnected=off
  tag scope: ASMBUS_Environment_Traffic_SamplePulse=scoped, ASMBUS_Environment_Traffic_SensorScheduler=scoped
  wires:
  GetFellowPositionVector/1(Angle_Fellows[deg]) -> SampleAndHold/3(In3)
  Bus Selector6/1 -> GetFellowPositionVector/1(<FellowPositions>)  "<Traffic_Signals_toEnvironment>"
  Traffic_Signals/1 -> Bus Selector6/1, Bus Selector2/1, GetObjectSignals/1(Traffic_Signals), Bus Selector5/1
  GetFellowPositionVector/2(Pos_Fellows_MainPnt_CoorSys_E[x;y;z][m]) -> SampleAndHold/4(In4)
  SampleAndHold/6(Out6) -> OBJECT_SENSOR_3D_CALCULATION/10
  Bus Selector5/2 -> SampleAndHold/6(In6)  "<v_Fellows[x;y;z][km|h]>"
  Bus Selector1/1 -> Init_Ready[0Off|1On]/1
  Enable_Init[0Off|1On]/1 -> OBJECT_SENSOR_3D_CALCULATION/1
  OBJECT_SENSOR_3D_CALCULATION/3 -> SensorData[]/1
  Bus Selector4/1 -> OBJECT_SENSOR_3D_CALCULATION/15
  SENSOR_SCHEDULER/4 -> Mux/2
  Mux/1 -> OBJECT_SENSOR_3D_CALCULATION/2
  SENSOR_SCHEDULER/3 -> Terminator7/1
  SampleAndHold/4(Out4) -> OBJECT_SENSOR_3D_CALCULATION/8
  SampleAndHold/3(Out3) -> OBJECT_SENSOR_3D_CALCULATION/7
  SampleAndHold/5(Out5) -> OBJECT_SENSOR_3D_CALCULATION/9
  SampleAndHold/2(Out2) -> Pos_Vehicle_CoorSys_E_Sampled[x,y;z][m]/1, OBJECT_SENSOR_3D_CALCULATION/6
  SampleAndHold/1(Out1) -> Angle_Vehicle_CoorSys_E_Sampled[x,y;z][deg]/1, OBJECT_SENSOR_3D_CALCULATION/5
  SENSOR_SCHEDULER/9 -> Terminator4/1
  SENSOR_SCHEDULER/5 -> OBJECT_SENSOR_3D_CALCULATION/3
  Bus Selector5/1 -> SampleAndHold/5(In5)  "<Flag_FellowUsed[0|1]>"
  SENSOR_SCHEDULER/2 -> SensorMapping_Data[]/1
  SENSOR_SCHEDULER/6 -> OBJECT_SENSOR_3D_PARAM_SELECTION/1
  Bus to Vector/1 -> OBJECT_SENSOR_3D_CALCULATION/12
  Interface_In/1 -> Bus Selector/1
  Road_Signals/1 -> Bus Selector4/1
  Bus Selector/2 -> SampleAndHold/2(In2)  "<Pos_Vehicle_CoorSys_E[x;y;z][m]>"
  Bus Selector/1 -> SampleAndHold/1(In1)  "<Angle_Vehicle_CoorSys_E[x;y;z][deg]>"
  GetObjectSignals/1(PosVec_MainPnt_Fellows[x;y;z][m]) -> OBJECT_SENSOR_3D_CALCULATION/11
  Sensor_Data[]/1 -> OBJECT_SENSOR_3D_PARAM_VECTORIZATION/1
  Enable[0Off|1On]/1 -> SAMPLE_PULSE/1, Mux/1, SENSOR_SCHEDULER/1
  SENSOR_SCHEDULER/7 -> Terminator2/1
  OBJECT_SENSOR_3D_CALCULATION/1 -> Terminator3/1
  OBJECT_SENSOR_3D_PARAM_SELECTION/1 -> OBJECT_SENSOR_3D_CALCULATION/4
  SENSOR_SCHEDULER/8 -> Terminator1/1
  OBJECT_SENSOR_3D_CALCULATION/2 -> SensorSignals/1, Bus Selector1/1
  SENSOR_SCHEDULER/1 -> [ASMBUS_Environment_Traffic_SensorScheduler]
  OBJECT_SENSOR_3D_PARAM_VECTORIZATION/1 -> SENSOR_SCHEDULER/2
  OBJECT_SENSOR_3D_PARAM_VECTORIZATION/2 -> OBJECT_SENSOR_3D_PARAM_SELECTION/2
  SAMPLE_PULSE/2 -> SampleAndHold/Enable
  SAMPLE_PULSE/1 -> [ASMBUS_Environment_Traffic_SamplePulse]
  Bus Selector2/1 -> OBJECT_SENSOR_3D_CALCULATION/16  "<TrafficObjectsState[]>"
  GetObjectSignals/2(Size_Fellows[m]) -> Bus to Vector/1
  GetObjectSignals/3(TrafficObject_Type_Data[]) -> OBJECT_SENSOR_3D_CALCULATION/13
  GetObjectSignals/4(TrafficObject_Type_Fellows[]) -> OBJECT_SENSOR_3D_CALCULATION/14
  Sensor_Time_Base[s]/1 -> SampleAndHold/7(In7), OBJECT_SENSOR_3D_CALCULATION/18
  SampleAndHold/7(Out7) -> OBJECT_SENSOR_3D_CALCULATION/17

== system ASM_Traffic/Environment/Sensors/PlantModel/Object_Sensor_3D/SensorMapping ==
  Enable[0Off|1On] : Inport
  SensorMapping_Data[] : Inport  Port=2
  SensorSignals : Inport  Port=3
  Bus Creator : BusCreator  Inputs=3
  Demux : Demux  Outputs=[4,4,4]
  OBJECT_SENSOR_3D_MAPPING1 : ASM_Traffic_lib/Sensors/Object_Sensor_3D/OBJECT_SENSOR_3D_MAPPING  ASMProperties=struct('Name','OBJECT_SENSOR_3D_MAPPING','Version','10.0','Library','ASM_Traffic_lib')  ASMInstanceName=object_sensor_3d_mapping  ASMInstanceID=1
  OBJECT_SENSOR_3D_MAPPING2 : ASM_Traffic_lib/Sensors/Object_Sensor_3D/OBJECT_SENSOR_3D_MAPPING  ASMProperties=struct('Name','OBJECT_SENSOR_3D_MAPPING','Version','10.0','Library','ASM_Traffic_lib')  ASMInstanceName=object_sensor_3d_mapping  ASMInstanceID=1
  OBJECT_SENSOR_3D_MAPPING3 : ASM_Traffic_lib/Sensors/Object_Sensor_3D/OBJECT_SENSOR_3D_MAPPING  ASMProperties=struct('Name','OBJECT_SENSOR_3D_MAPPING','Version','10.0','Library','ASM_Traffic_lib')  ASMInstanceName=object_sensor_3d_mapping  ASMInstanceID=1
  Signals_ASMSignalCollector : Subsystem
  Signals_to_ACC_SoftECU : Subsystem
  Sensor_Signals : Outport  VectorParamsAs1DForOutWhenUnconnected=off
  tag scope: ASMBUS_Environment_Traffic_3DObjSensor_SensorSignals=scoped, ASMBUS_Environment_Traffic_3DObjSensor_SensorSignals_Status=scoped
  wires:
  Bus Creator/1 -> [ASMBUS_Environment_Traffic_3DObjSensor_SensorSignals]
  Signals_ASMSignalCollector/1(Sfcn_Status) -> [ASMBUS_Environment_Traffic_3DObjSensor_SensorSignals_Status]  "Sfcn_Status"
  SensorSignals/1 -> OBJECT_SENSOR_3D_MAPPING1/3, OBJECT_SENSOR_3D_MAPPING2/3, OBJECT_SENSOR_3D_MAPPING3/3, Signals_ASMSignalCollector/1(SensorSignals)
  Enable[0Off|1On]/1 -> OBJECT_SENSOR_3D_MAPPING1/1, OBJECT_SENSOR_3D_MAPPING3/1, OBJECT_SENSOR_3D_MAPPING2/1
  Demux/2 -> OBJECT_SENSOR_3D_MAPPING2/2
  OBJECT_SENSOR_3D_MAPPING3/1 -> Bus Creator/3  "Sensor3"
  OBJECT_SENSOR_3D_MAPPING2/1 -> Signals_to_ACC_SoftECU/2(Sensor_2_ACC_In), Bus Creator/2  "Sensor2"
  SensorMapping_Data[]/1 -> Demux/1
  Signals_to_ACC_SoftECU/1(Sensor_Signals) -> Sensor_Signals/1
  OBJECT_SENSOR_3D_MAPPING1/1 -> Signals_to_ACC_SoftECU/1(Sensor_1_ACC_In), Bus Creator/1  "Sensor1"
  Demux/3 -> OBJECT_SENSOR_3D_MAPPING3/2
  Demux/1 -> OBJECT_SENSOR_3D_MAPPING1/2

== system ASM_Traffic/Environment/Sensors/PlantModel/Object_Sensor_3D/SensorParameters ==
  ObjectSensor3DParameters_1 : Subsystem
  ObjectSensor3DParameters_2 : Subsystem
  ObjectSensor3DParameters_3 : Subsystem
  Vector Concatenate : Concatenate  NumInputs=3  Mode=Multidimensional array  ConcatenateDimension=2
  Sensor_Data[] : Outport  VectorParamsAs1DForOutWhenUnconnected=off
  wires:
  ObjectSensor3DParameters_3/1(Sensor_Parameters[]) -> Vector Concatenate/3
  ObjectSensor3DParameters_2/1(Sensor_Parameters[]) -> Vector Concatenate/2
  ObjectSensor3DParameters_1/1(Sensor_Parameters[]) -> Vector Concatenate/1
  Vector Concatenate/1 -> Sensor_Data[]/1

== system ASM_Traffic/Environment/Sensors/PlantModel/Sensors_Common_Signals/Enable_Scheduling ==
  Enable_In[0Off|1On] : Inport
  Constant : Constant  Value=0.5  SampleTime=-1
  Constant1 : Constant  SampleTime=-1
  Constant2 : Constant  Value=0  SampleTime=-1
  Enable_Sensor : Gain
  Multiport Switch : MultiPortSwitch  DataPortOrder=Zero-based contiguous  Inputs=2  zeroidx=on  SaturateOnIntegerOverflow=off  InputSameDT=off
  Relational Operator : RelationalOperator  Operator=>  OutDataTypeStr=boolean  InputSameDT=off
  Enable_Out[0Off|1On] : Outport  VectorParamsAs1DForOutWhenUnconnected=off
  wires:
  Constant2/1 -> Multiport Switch/2
  Constant1/1 -> Multiport Switch/3
  Constant/1 -> Relational Operator/2
  Multiport Switch/1 -> Enable_Out[0Off|1On]/1
  Relational Operator/1 -> Multiport Switch/1
  Enable_Sensor/1 -> Relational Operator/1
  Enable_In[0Off|1On]/1 -> Enable_Sensor/1

== system ASM_Traffic/Environment/Sensors/PlantModel/Sensors_Common_Signals/Maneuver_Start ==
  ManeuverState_Change[0|1] : Inport
  Detect Change : simulink/Logic and Bit Operations/Detect Change  vinit=0  OutDataTypeStr=boolean
  Digital Clock : DigitalClock  SampleTime=SIM.StepSize.v
  Memory1 : Memory
  Multiport Switch : MultiPortSwitch  DataPortOrder=Zero-based contiguous  Inputs=2  zeroidx=on  SaturateOnIntegerOverflow=off  InputSameDT=off
  Product : Product
  Product1 : Product
  Product2 : Product
  ManeuverStart[s] : Outport
  wires:
  Product/1 -> ManeuverStart[s]/1
  Digital Clock/1 -> Multiport Switch/3
  Detect Change/1 -> Product1/2
  Product1/1 -> Multiport Switch/1
  ManeuverState_Change[0|1]/1 -> Product1/1, Detect Change/1, Product/2, Product2/1
  Memory1/1 -> Product2/2
  Product2/1 -> Multiport Switch/2
  Multiport Switch/1 -> Memory1/1, Product/1

== system ASM_Traffic/Environment/Sensors/PlantModel/Sensors_Common_Signals/Sensor_Init_Trigger ==
  DiscreteObjects_Data_Valid[] : Inport
  Constant1 : Constant
  Constant2 : Constant  Value=0
  Constant5 : Constant
  Constant6 : Constant  Value=0
  Data Type Conversion : DataTypeConversion  OutDataTypeStr=double  SaturateOnIntegerOverflow=off  RndMeth=Floor
  Enable_Sensor_Init : Gain
  Logical Operator : Logic  AllPortsSameDT=off
  Memory : UnitDelay  SampleTime=-1
  Relational Operator : RelationalOperator  Operator===
  Relational Operator1 : RelationalOperator  Operator===
  Start : MultiPortSwitch  DataPortOrder=Zero-based contiguous  Inputs=2  zeroidx=on  InputSameDT=off
  Ctrl : Outport  VectorParamsAs1DForOutWhenUnconnected=off
  wires:
  Enable_Sensor_Init/1 -> Start/1
  Data Type Conversion/1 -> Relational Operator/1, Memory/1
  DiscreteObjects_Data_Valid[]/1 -> Data Type Conversion/1
  Memory/1 -> Relational Operator1/1
  Constant1/1 -> Relational Operator/2
  Constant2/1 -> Relational Operator1/2
  Relational Operator/1 -> Logical Operator/1
  Relational Operator1/1 -> Logical Operator/2
  Logical Operator/1 -> Enable_Sensor_Init/1
  Constant6/1 -> Start/2
  Constant5/1 -> Start/3
  Start/1 -> Ctrl/1  "start"

== system ASM_Traffic/Environment/Sensors/PlantModel/Sensors_Common_Signals/Sensor_Time_Base ==
  ManeuverState_Change[0|1] : Inport
  ManeuverStart[s] : Inport  Port=2
  Add : Sum  Inputs=-+
  Digital Clock : DigitalClock  SampleTime=SIM.StepSize.v
  Product3 : Product
  Sensor_Time_Base[s] : Outport
  wires:
  ManeuverStart[s]/1 -> Add/1
  Add/1 -> Product3/1
  Product3/1 -> Sensor_Time_Base[s]/1
  Digital Clock/1 -> Add/2
  ManeuverState_Change[0|1]/1 -> Product3/2

== system ASM_Traffic/Environment/Sensors/PlantModel/Sensors_Common_Signals/SignalCollector ==
  ManeuverStart[s] : Inport
  Enable_SensorScheduling[0Off|1On] : Inport  Port=2
  Init_Ready[0Off|1On] : Inport  Port=3
  Bus Creator2 : BusCreator  Inputs=3
  ASMSignalBus : Outport  VectorParamsAs1DForOutWhenUnconnected=off
  wires:
  Init_Ready[0Off|1On]/1 -> Bus Creator2/3  "Sensor_Init_Ready[0Off|1On]"
  Enable_SensorScheduling[0Off|1On]/1 -> Bus Creator2/2  "Enable_SensorScheduling[0Off|1On]"
  Bus Creator2/1 -> ASMSignalBus/1  "Sensors_Common"
  ManeuverStart[s]/1 -> Bus Creator2/1  "ManeuverStart[s]"

== system ASM_Traffic/Environment/Sensors/PlantModel/Traffic_Sign_Sensor/ASMSignalCollector ==
  Bus Creator1 : BusCreator  Inputs=3
  Bus Creator2 : BusCreator  Inputs=1
  Bus Selector : BusSelector  OutputSignals=Info,SensorOutput[]
  tag scope: ASMBUS_Environment_Traffic_Sensors_Traffic_Sign_Sensor_dyn=scoped
  wires:
  Bus Creator2/1 -> [ASMBUS_Environment_Traffic_Sensors_Traffic_Sign_Sensor_dyn]  "TrafficSign_Sensor_Dyn"
  Bus Creator1/1 -> Bus Creator2/1  "Sensor_Front_1"
  Bus Selector/2 -> Bus Creator1/2  "<SensorOutput[]>"
  Bus Selector/1 -> Bus Creator1/1  "<Info>"
  [ASMBUS_Traf_Sensors_Traffic_Sign_Sensor_dyn_1_Parameters] -> Bus Creator1/3  "Parameters"
  [ASMBUS_Traf_Sensors_dyn_Traffic_Sign_Sensor_1] -> Bus Selector/1

== system ASM_Traffic/Environment/Sensors/PlantModel/Traffic_Sign_Sensor/Enable_Traffic_Sign_Sensor ==
  Enable_In[0Off|1On] : Inport
  Constant : Constant  Value=0.5  SampleTime=-1
  Constant1 : Constant  SampleTime=-1
  Constant2 : Constant  Value=0  SampleTime=-1
  Enable_Sensor : Gain
  Multiport Switch : MultiPortSwitch  DataPortOrder=Zero-based contiguous  Inputs=2  zeroidx=on  SaturateOnIntegerOverflow=off  InputSameDT=off
  Relational Operator : RelationalOperator  Operator=>  OutDataTypeStr=boolean  InputSameDT=off
  Enable_Out[0Off|1On] : Outport  VectorParamsAs1DForOutWhenUnconnected=off
  wires:
  Constant2/1 -> Multiport Switch/2
  Constant1/1 -> Multiport Switch/3
  Constant/1 -> Relational Operator/2
  Multiport Switch/1 -> Enable_Out[0Off|1On]/1
  Relational Operator/1 -> Multiport Switch/1
  Enable_Sensor/1 -> Relational Operator/1
  Enable_In[0Off|1On]/1 -> Enable_Sensor/1

== system ASM_Traffic/Environment/Sensors/PlantModel/Traffic_Sign_Sensor/Objects_DataStreams ==
  TrafficObjects_States_In[] : Inport
  Bus Selector : BusSelector  OutputSignals=DataStream_1[].DataStream_1[],DataStream_2[].DataStream_2[],DataStream_3[].DataStream_3[],DataStream_4[].DataStream_4[],DataStream_5[].DataStream_5[],DataStream_6[].DataStream_6[],DataStream_7[].DataStream_7[],DataStream_8[].DataStream_8[]
  Mux : Mux  Inputs=8
  TrafficObjects_States[] : Outport  VectorParamsAs1DForOutWhenUnconnected=off
  wires:
  TrafficObjects_States_In[]/1 -> Bus Selector/1
  Bus Selector/8 -> Mux/8  "<DataStream_8[]>"
  Bus Selector/7 -> Mux/7  "<DataStream_7[]>"
  Bus Selector/6 -> Mux/6  "<DataStream_6[]>"
  Bus Selector/5 -> Mux/5  "<DataStream_5[]>"
  Bus Selector/4 -> Mux/4  "<DataStream_4[]>"
  Bus Selector/3 -> Mux/3  "<DataStream_3[]>"
  Bus Selector/2 -> Mux/2  "<DataStream_2[]>"
  Bus Selector/1 -> Mux/1  "<DataStream_1[]>"
  Mux/1 -> TrafficObjects_States[]/1

== system ASM_Traffic/Environment/Sensors/UserInterface/DISP_Plant/Line_Sensor ==
  note: LineSensor-Output not
      | fed into SignalBus due
      | to large amount of signal data.
  TrafficBus : Inport
  Bus Selector : BusSelector  OutputSignals=Line_Sensor.Line_Sensor_1.Info
  Bus Selector1 : BusSelector  OutputSignals=LineSensor_Data_Valid[0|1|2],Num_Pnts_Detected_Road_Lanes[],Num_Pnts_Detected_Road_Shape_Lines[],Num_Pnts_Detected_Road_Shape_ContObj[],Num_Pnts_Detected_Junction_Borders[],Num_Pnts_Detected_Junction_Shape_Lines[],Num_Pnts_Detected_Junction_Shape_ContObj[]
  Data_Valid[0|1|2] : Subsystem
      mask Display: disp('')
  Line_Sensor_Info : Scope  NumInputPorts=7
      settings: TimeSpan=5  ActiveDisplayYMinimum=1  ActiveDisplayYMaximum=2  DataLoggingMaxPoints=20000  DataLoggingDecimation=10  DataLoggingVariableName=ScopeData30
  Num_Pnts_Detected_Junction_Borders[] : Subsystem
      mask Display: disp('')
  Num_Pnts_Detected_Junction_Shape_ContObj[] : Subsystem
      mask Display: disp('')
  Num_Pnts_Detected_Junction_Shape_Lines[] : Subsystem
      mask Display: disp('')
  Num_Pnts_Detected_Road_Lanes[] : Subsystem
      mask Display: disp('')
  Num_Pnts_Detected_Road_Shape_ContObj[] : Subsystem
      mask Display: disp('')
  Num_Pnts_Detected_Road_Shape_Lines[] : Subsystem
      mask Display: disp('')
  wires:
  Num_Pnts_Detected_Junction_Shape_ContObj[]/1(Out1) -> Line_Sensor_Info/7  "Num_Pnts_Detected_Junction_Shape_ContObj[]"
  Num_Pnts_Detected_Junction_Shape_Lines[]/1(Out1) -> Line_Sensor_Info/6  "Num_Pnts_Detected_Junction_Shape_Lines[]"
  Bus Selector1/6 -> Num_Pnts_Detected_Junction_Shape_Lines[]/1(In1)  "<Num_Pnts_Detected_Junction_Shape_Lines[]>"
  Bus Selector1/7 -> Num_Pnts_Detected_Junction_Shape_ContObj[]/1(In1)  "<Num_Pnts_Detected_Junction_Shape_ContObj[]>"
  Num_Pnts_Detected_Junction_Borders[]/1(Out1) -> Line_Sensor_Info/5  "Num_Pnts_Detected_Junction_Borders[]"
  Bus Selector1/5 -> Num_Pnts_Detected_Junction_Borders[]/1(In1)  "<Num_Pnts_Detected_Junction_Borders[]>"
  Num_Pnts_Detected_Road_Shape_ContObj[]/1(Out1) -> Line_Sensor_Info/4  "Num_Pnts_Detected_Road_Shape_ContObj[]"
  Bus Selector1/4 -> Num_Pnts_Detected_Road_Shape_ContObj[]/1(In1)  "<Num_Pnts_Detected_Road_Shape_ContObj[]>"
  Bus Selector/1 -> Bus Selector1/1  "<Info>"
  Bus Selector1/1 -> Data_Valid[0|1|2]/1(In1)  "<LineSensor_Data_Valid[0|1|2]>"
  Bus Selector1/2 -> Num_Pnts_Detected_Road_Lanes[]/1(In1)  "<Num_Pnts_Detected_Road_Lanes[]>"
  Data_Valid[0|1|2]/1(Out1) -> Line_Sensor_Info/1  "Data_Valid[0|1|2]"
  Num_Pnts_Detected_Road_Lanes[]/1(Out1) -> Line_Sensor_Info/2  "Num_Pnts_Detected_Road_Lanes[]"
  Bus Selector1/3 -> Num_Pnts_Detected_Road_Shape_Lines[]/1(In1)  "<Num_Pnts_Detected_Road_Shape_Lines[]>"
  Num_Pnts_Detected_Road_Shape_Lines[]/1(Out1) -> Line_Sensor_Info/3  "Num_Pnts_Detected_Road_Shape_Lines[]"
  TrafficBus/1 -> Bus Selector/1
